simulink model "quadrotor_6dof_flight"  (R2025b)
settings: Solver=ode4  StartTime=0.0  StopTime=10.0  FixedStep=1e-3  RelTol=1e-3
settings Model: Creator=user  LastModifiedBy=user

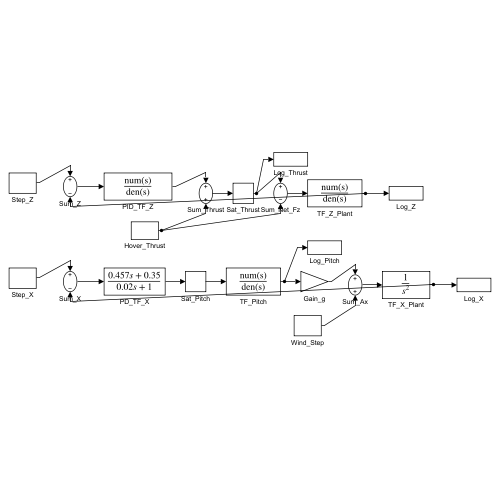
[thumbnail: Simulink's stored preview of the top-level diagram]
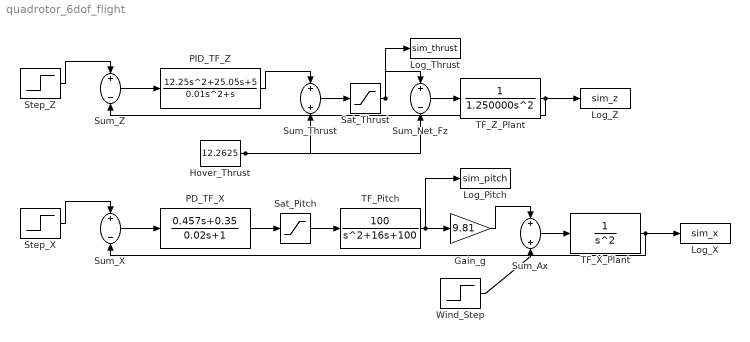
== system quadrotor_6dof_flight ==
  Gain_g : Gain  Gain=9.81
  Hover_Thrust : Constant  Value=12.2625
  Log_Pitch : ToWorkspace  VariableName=sim_pitch  SampleTime=-1
  Log_Thrust : ToWorkspace  VariableName=sim_thrust  SampleTime=-1
  Log_X : ToWorkspace  VariableName=sim_x  SampleTime=-1
  Log_Z : ToWorkspace  VariableName=sim_z  SampleTime=-1
  PD_TF_X : TransferFcn  Numerator=[0.457 0.35]  Denominator=[0.02 1]
  PID_TF_Z : TransferFcn  Numerator=[12.25 25.05 5]  Denominator=[0.01 1 0]
  Sat_Pitch : Saturate  UpperLimit=0.35  LowerLimit=-0.35
  Sat_Thrust : Saturate  UpperLimit=36  LowerLimit=0
  Step_X : Step  Time=2.0  After=3  SampleTime=0
  Step_Z : Step  Time=0.5  After=5  SampleTime=0
  Sum_Ax : Sum
  Sum_Net_Fz : Sum  Inputs=+-
  Sum_Thrust : Sum
  Sum_X : Sum  Inputs=+-
  Sum_Z : Sum  Inputs=+-
  TF_Pitch : TransferFcn  Numerator=[100]  Denominator=[1 16 100]
  TF_X_Plant : TransferFcn  Denominator=[1 0 0]
  TF_Z_Plant : TransferFcn  Denominator=[1.250000 0 0]
  Wind_Step : Step  Time=5.0  After=-0.8  SampleTime=0
  wires:
  Step_Z/1 -> Sum_Z/1
  Sum_Z/1 -> PID_TF_Z/1
  PID_TF_Z/1 -> Sum_Thrust/1
  Hover_Thrust/1 -> Sum_Thrust/2, Sum_Net_Fz/2
  Sum_Thrust/1 -> Sat_Thrust/1
  Sat_Thrust/1 -> Sum_Net_Fz/1, Log_Thrust/1
  Sum_Net_Fz/1 -> TF_Z_Plant/1
  TF_Z_Plant/1 -> Sum_Z/2, Log_Z/1
  Step_X/1 -> Sum_X/1
  Sum_X/1 -> PD_TF_X/1
  PD_TF_X/1 -> Sat_Pitch/1
  Sat_Pitch/1 -> TF_Pitch/1
  TF_Pitch/1 -> Gain_g/1, Log_Pitch/1
  Gain_g/1 -> Sum_Ax/1
  Wind_Step/1 -> Sum_Ax/2
  Sum_Ax/1 -> TF_X_Plant/1
  TF_X_Plant/1 -> Sum_X/2, Log_X/1
